simulink model "NBMS_DischargeOCV"  (R2026b)
settings: Solver=FixedStepDiscrete  StopTime=20  FixedStep=0.1
undefined symbols (not defined in the file): X_SOC_VS_OCV_DISCH, Y_SOC_VS_OCV_DISCH
settings Model: Creator=hp  LastModifiedBy=rathi
settings OptimizationCC: DefaultParameterBehavior=Inlined  DifferentSizesBufferReuse=on  EfficientTunableParamExpr=on  EnhancedBackFolding=on  OptimizationCustomize=off  OptimizeBlockOrder=speed  PassReuseOutputArgsAs=Individual arguments  RemoveInternalMemoryZeroInit=on  RemoveRootLevelIOMemoryZeroInit=on
settings DebuggingCC: ParameterTunabilityLossMsg=error
settings SFSimCC: MATLABDynamicMemAlloc=off
settings RTWCC: Description=Embedded Coder  GenCodeOnly=on  PackageGeneratedCodeAndArtifacts=on  SystemTargetFile=ert.tlc  TemplateMakefile=ert_default_tmf
settings CodeAppCC: ForceParamTrailComments=on  IgnoreCustomStorageClasses=off  InsertBlockDesc=on  OperatorAnnotations=on  SFDataObjDesc=on  SimulinkDataObjDesc=on
settings ERTTargetCC: DynamicArrayContainerType=coder::array  GenerateSampleERTMain=on
settings ConfigComp: DVDefectChecker=on  DVDetectOutOfBounds=on  DVHarnessSource=Signal Editor  DVModelReferenceHarness=on  DVTestSuiteOptimization=Auto

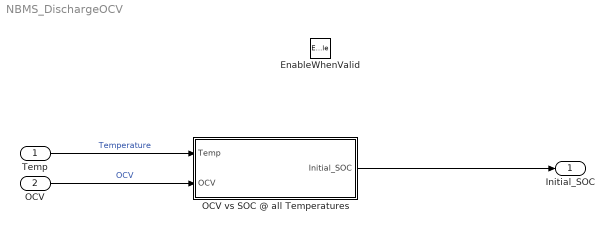
== system NBMS_DischargeOCV ==
  Temp : Inport
  OCV : Inport  Port=2  OutDataTypeStr=fixdt(1,16,0.001,0)
  EnableWhenValid : EnablePort  StatesWhenEnabling=reset  OutDataTypeStr=boolean
  OCV vs SOC @ all Temperatures : Subsystem  TreatAsAtomicUnit=on
  Initial_SOC : Outport  OutputWhenDisabled=reset  InitialOutput=0
  wires:
  OCV/1 -> OCV vs SOC @ all Temperatures/2(OCV)  "OCV"
  Temp/1 -> OCV vs SOC @ all Temperatures/1(Temp)  "Temperature"
  OCV vs SOC @ all Temperatures/1(Initial_SOC) -> Initial_SOC/1

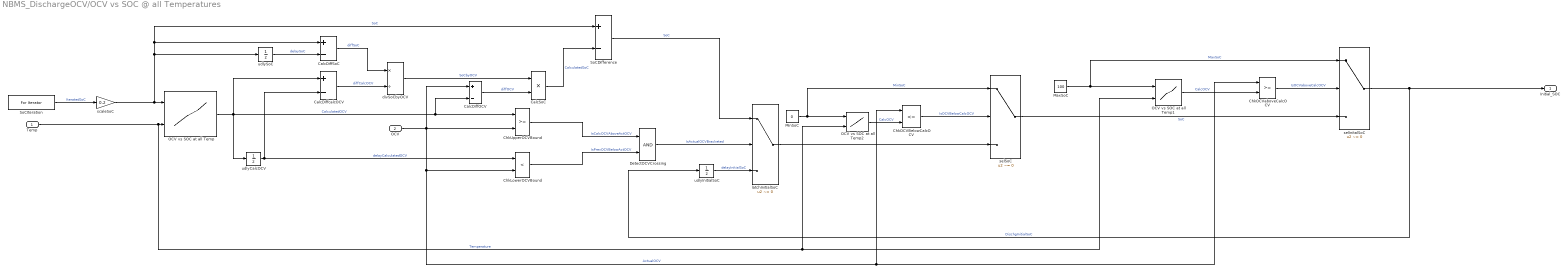
== system NBMS_DischargeOCV/OCV vs SOC @ all Temperatures ==
  Temp : Inport
  OCV : Inport  Port=2
  CalcDiffOCV : Sum  Inputs=+-
  CalcDiffSoC : Sum  Inputs=+-
  CalcDiffcalcOCV : Sum  Inputs=+-
  CalcSoC : Product
  ChkLowerOCVBound : RelationalOperator  Operator=<  OutDataTypeStr=boolean  RndMeth=Simplest  InputSameDT=off
  ChkOCVBelowCalcOCV : RelationalOperator  Operator=<=  OutDataTypeStr=boolean  RndMeth=Simplest  InputSameDT=off
  ChkOCVaboveCalcOCV : RelationalOperator  OutDataTypeStr=boolean  RndMeth=Simplest  InputSameDT=off
  ChkUpperOCVBound : RelationalOperator  OutDataTypeStr=boolean  RndMeth=Simplest  InputSameDT=off
  DetectOCVCrossing : Logic  AllPortsSameDT=off  OutDataTypeStr=boolean
  MaxSoC : Constant  Value=100
  MinSoC : Constant  Value=0
  OCV vs SOC at all Temp : Lookup_n-D  BreakpointsForDimension1=X_SOC_VS_OCV_DISCH  BreakpointsForDimension2=Y_SOC_VS_OCV_DISCH  BreakpointsForDimension1DataTypeStr=double  BreakpointsForDimension2DataTypeStr=double  Table=[2.934 2.929 2.92 2.9 2.911 2.903 2.922;3.148 3.135 3.129 3.118 3.123 3.121 3.133;3.295 3.294 3.289 3.281 3.272 3.266 3.276;3.409 3.409 3.405 3.4 3.395 3.386 3.395;3.45 3.452 3.451 3.451 3.452 3.449 3.452;3.494 3.501 3.501 3.499 3.499 3.49 3.496;3.552 3.559 3.558 3.557 3.554 3.546 3.551;3.597 3.607 3.607 3.606 3.603 3.593 3.598;3.636 3.64 3.641 3.642 3.642 3.642 3.648;3.667 3.672 3.674 3.676 3.676 3.679 3.685;3.708 3.715 3.717 3.718 3.718 3.721 3.727;3.753 3.756 3.758 3.759 3.763 3.766 3.763;3.799 3.803 3.805 3.807 3.813 3.812 3.808;3.868 3.872 3.872 3.87 3.877 3.874 3.866;3.907 3.909 3.91 3.91 3.912 3.911 3.907;3.946 3.949 3.95 3.95 3.953 3.952 3.947;4.006 4.008 4.009 4.009 4.012 4.011 4.005;4.057 4.059 4.06 4.06 4.063 4.063 4.059;4.072 4.075 4.077 4.077 4.08 4.08 4.079;4.087 4.091 4.093 4.094 4.096 4.096 4.094;4.185 4.185 4.185 4.185 4.185 4.185 4.185]  TableDataTypeStr=double  IntermediateResultsDataTypeStr=double  ExtrapMethod=Clip  OutDataTypeStr=double  RndMeth=Simplest  SaturateOnIntegerOverflow=on  FractionDataTypeStr=double
      settings: InputPortMap=u0,u1
  OCV vs SOC at all Temp1 : Lookup_n-D  BreakpointsForDimension1=X_SOC_VS_OCV_DISCH  BreakpointsForDimension2=Y_SOC_VS_OCV_DISCH  BreakpointsForDimension1DataTypeStr=double  BreakpointsForDimension2DataTypeStr=double  Table=[2.934 2.929 2.92 2.9 2.911 2.903 2.922;3.148 3.135 3.129 3.118 3.123 3.121 3.133;3.295 3.294 3.289 3.281 3.272 3.266 3.276;3.409 3.409 3.405 3.4 3.395 3.386 3.395;3.45 3.452 3.451 3.451 3.452 3.449 3.452;3.494 3.501 3.501 3.499 3.499 3.49 3.496;3.552 3.559 3.558 3.557 3.554 3.546 3.551;3.597 3.607 3.607 3.606 3.603 3.593 3.598;3.636 3.64 3.641 3.642 3.642 3.642 3.648;3.667 3.672 3.674 3.676 3.676 3.679 3.685;3.708 3.715 3.717 3.718 3.718 3.721 3.727;3.753 3.756 3.758 3.759 3.763 3.766 3.763;3.799 3.803 3.805 3.807 3.813 3.812 3.808;3.868 3.872 3.872 3.87 3.877 3.874 3.866;3.907 3.909 3.91 3.91 3.912 3.911 3.907;3.946 3.949 3.95 3.95 3.953 3.952 3.947;4.006 4.008 4.009 4.009 4.012 4.011 4.005;4.057 4.059 4.06 4.06 4.063 4.063 4.059;4.072 4.075 4.077 4.077 4.08 4.08 4.079;4.087 4.091 4.093 4.094 4.096 4.096 4.094;4.185 4.185 4.185 4.185 4.185 4.185 4.185]  TableDataTypeStr=double  IntermediateResultsDataTypeStr=double  ExtrapMethod=Clip  OutDataTypeStr=double  RndMeth=Simplest  SaturateOnIntegerOverflow=on  FractionDataTypeStr=double
      settings: InputPortMap=u0,u1
  OCV vs SOC at all Temp2 : Lookup_n-D  BreakpointsForDimension1=X_SOC_VS_OCV_DISCH  BreakpointsForDimension2=Y_SOC_VS_OCV_DISCH  BreakpointsForDimension1DataTypeStr=double  BreakpointsForDimension2DataTypeStr=double  Table=[2.934 2.929 2.92 2.9 2.911 2.903 2.922;3.148 3.135 3.129 3.118 3.123 3.121 3.133;3.295 3.294 3.289 3.281 3.272 3.266 3.276;3.409 3.409 3.405 3.4 3.395 3.386 3.395;3.45 3.452 3.451 3.451 3.452 3.449 3.452;3.494 3.501 3.501 3.499 3.499 3.49 3.496;3.552 3.559 3.558 3.557 3.554 3.546 3.551;3.597 3.607 3.607 3.606 3.603 3.593 3.598;3.636 3.64 3.641 3.642 3.642 3.642 3.648;3.667 3.672 3.674 3.676 3.676 3.679 3.685;3.708 3.715 3.717 3.718 3.718 3.721 3.727;3.753 3.756 3.758 3.759 3.763 3.766 3.763;3.799 3.803 3.805 3.807 3.813 3.812 3.808;3.868 3.872 3.872 3.87 3.877 3.874 3.866;3.907 3.909 3.91 3.91 3.912 3.911 3.907;3.946 3.949 3.95 3.95 3.953 3.952 3.947;4.006 4.008 4.009 4.009 4.012 4.011 4.005;4.057 4.059 4.06 4.06 4.063 4.063 4.059;4.072 4.075 4.077 4.077 4.08 4.08 4.079;4.087 4.091 4.093 4.094 4.096 4.096 4.094;4.185 4.185 4.185 4.185 4.185 4.185 4.185]  TableDataTypeStr=double  IntermediateResultsDataTypeStr=double  ExtrapMethod=Clip  OutDataTypeStr=double  RndMeth=Simplest  SaturateOnIntegerOverflow=on  FractionDataTypeStr=double
      settings: InputPortMap=u0,u1
  SoCDifference : Sum  Inputs=+-
  SoCIteration : ForIterator  ResetStates=reset  IterationLimit=501  IndexMode=Zero-based  IterationVariableDataType=double
  divSoCbyOCV : Product  Inputs=*/
  latchInitialSoC : Switch  Criteria=u2 ~= 0  SaturateOnIntegerOverflow=off  InputSameDT=off
  scaleSoC : Gain  Gain=0.2
  selInitalSoC : Switch  Criteria=u2 ~= 0  SaturateOnIntegerOverflow=off  InputSameDT=off
  selSoC : Switch  Criteria=u2 ~= 0  SaturateOnIntegerOverflow=off  InputSameDT=off
  udlyCalcOCV : UnitDelay  SampleTime=-1
  udlyInitialSoC : UnitDelay  SampleTime=-1
  udlySoC : UnitDelay  SampleTime=-1
  Initial_SOC : Outport
  wires:
  scaleSoC/1 -> SoCDifference/1, CalcDiffSoC/1, udlySoC/1, OCV vs SOC at all Temp/1  "SoC"
  MinSoC/1 -> selSoC/1, OCV vs SOC at all Temp2/1  "MinSoC"
  OCV vs SOC at all Temp2/1 -> ChkOCVBelowCalcOCV/2  "CalcOCV"
  ChkOCVBelowCalcOCV/1 -> selSoC/2  "IsOCVBelowCalcOCV"
  latchInitialSoC/1 -> selSoC/3
  selInitalSoC/1 -> udlyInitialSoC/1, Initial_SOC/1  "DischgInitialSoC"
  selSoC/1 -> selInitalSoC/3  "SoC"
  MaxSoC/1 -> selInitalSoC/1, OCV vs SOC at all Temp1/1  "MaxSoC"
  OCV vs SOC at all Temp1/1 -> ChkOCVaboveCalcOCV/2  "CalcOCV"
  ChkOCVaboveCalcOCV/1 -> selInitalSoC/2  "IsOCVaboveCalcOCV"
  OCV/1 -> ChkOCVaboveCalcOCV/1, ChkOCVBelowCalcOCV/1, ChkLowerOCVBound/2, ChkUpperOCVBound/2, CalcDiffOCV/1  "ActualOCV"
  udlyCalcOCV/1 -> CalcDiffcalcOCV/2, ChkLowerOCVBound/1  "delayCalculatedOCV"
  SoCIteration/1 -> scaleSoC/1  "IteratedSoC"
  Temp/1 -> OCV vs SOC at all Temp1/2, OCV vs SOC at all Temp2/2, OCV vs SOC at all Temp/2  "Temperature"
  udlySoC/1 -> CalcDiffSoC/2  "delaySoC"
  OCV vs SOC at all Temp/1 -> ChkUpperOCVBound/1, CalcDiffOCV/2, CalcDiffcalcOCV/1, udlyCalcOCV/1  "CalculatedOCV"
  CalcDiffSoC/1 -> divSoCbyOCV/1  "diffSoC"
  CalcDiffOCV/1 -> CalcSoC/2  "diffOCV"
  CalcDiffcalcOCV/1 -> divSoCbyOCV/2  "diffCalcOCV"
  ChkLowerOCVBound/1 -> DetectOCVCrossing/2  "IsPrevOCVBelowActOCV"
  ChkUpperOCVBound/1 -> DetectOCVCrossing/1  "IsCalcOCVAboveActOCV"
  divSoCbyOCV/1 -> CalcSoC/1  "SoCbyOCV"
  DetectOCVCrossing/1 -> latchInitialSoC/2  "IsActualOCVBracketed"
  CalcSoC/1 -> SoCDifference/2  "CalculatedSoC"
  SoCDifference/1 -> latchInitialSoC/1  "SoC"
  udlyInitialSoC/1 -> latchInitialSoC/3  "delayInitialSoC"
